simulink model "EkfObserver"  (R2026b)
settings: Solver=VariableStepAuto
PostLoadFcn:
  | addpath(fullfile(fileparts(get_param(bdroot,'FileName')),'..','build_process'));initialize_ekf_paths();
undefined symbols (not defined in the file or in its folder): ekf_parameters
libraries: $bdroot x1
settings Model: Creator=24322  LastModifiedBy=24322

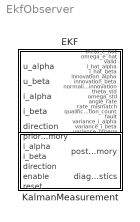
== system EkfObserver ==
  EKF : Subsystem  mask{cfg=ekf_parameters()}
      mask prompts: cfg "Kalman configuration"
  KalmanMeasurement : Subsystem  mask{cfg=ekf_parameters()}
      mask prompts: cfg "Kalman configuration"

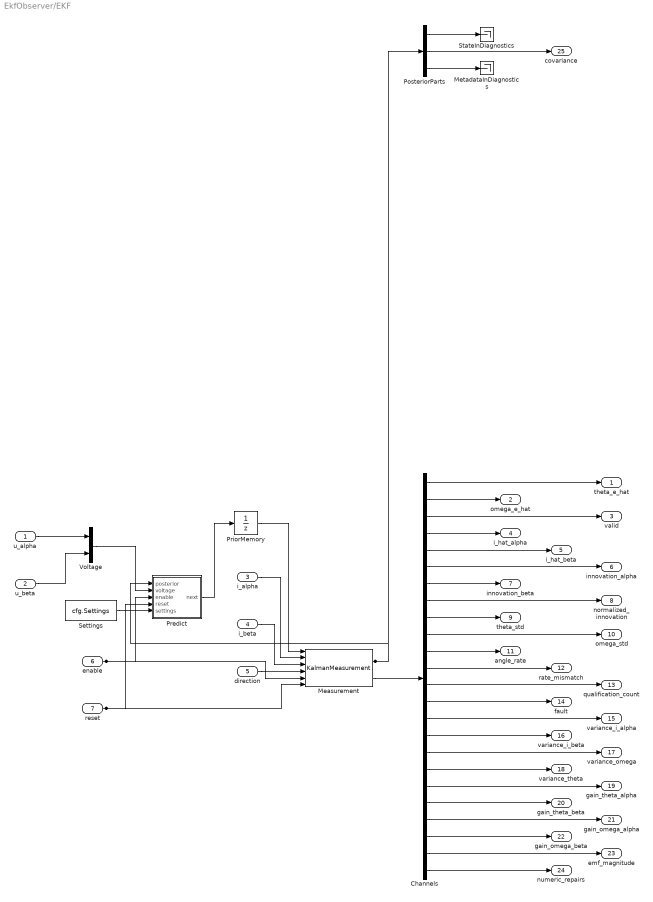
== system EkfObserver/EKF ==
  u_alpha : Inport  SampleTime=cfg.Model.Ts
  u_beta : Inport  Port=2  SampleTime=cfg.Model.Ts
  i_alpha : Inport  Port=3  SampleTime=cfg.Model.Ts
  i_beta : Inport  Port=4  SampleTime=cfg.Model.Ts
  direction : Inport  Port=5  SampleTime=cfg.Model.Ts
  enable : Inport  Port=6  SampleTime=cfg.Model.Ts
  reset : Inport  Port=7  SampleTime=cfg.Model.Ts
  Channels : Demux  Outputs=24
  Measurement : $bdroot/KalmanMeasurement  cfg=cfg
  MetadataInDiagnostics : Terminator
  PosteriorParts : Demux  Outputs=[4 16 8]
  Predict : MATLAB Function  TreatAsAtomicUnit=on
  PriorMemory : UnitDelay  InitialCondition=zeros(28,1)  SampleTime=cfg.Model.Ts
  Settings : Constant  Value=cfg.Settings
  StateInDiagnostics : Terminator
  Voltage : Mux  Inputs=2
  theta_e_hat : Outport
  omega_e_hat : Outport  Port=2
  valid : Outport  Port=3
  i_hat_alpha : Outport  Port=4
  i_hat_beta : Outport  Port=5
  innovation_alpha : Outport  Port=6
  innovation_beta : Outport  Port=7
  normalized_innovation : Outport  Port=8
  theta_std : Outport  Port=9
  omega_std : Outport  Port=10
  angle_rate : Outport  Port=11
  rate_mismatch : Outport  Port=12
  qualification_count : Outport  Port=13
  fault : Outport  Port=14
  variance_i_alpha : Outport  Port=15
  variance_i_beta : Outport  Port=16
  variance_omega : Outport  Port=17
  variance_theta : Outport  Port=18
  gain_theta_alpha : Outport  Port=19
  gain_theta_beta : Outport  Port=20
  gain_omega_alpha : Outport  Port=21
  gain_omega_beta : Outport  Port=22
  emf_magnitude : Outport  Port=23
  numeric_repairs : Outport  Port=24
  covariance : Outport  Port=25
  wires:
  Channels/24 -> numeric_repairs/1
  Channels/23 -> emf_magnitude/1
  Channels/22 -> gain_omega_beta/1
  Channels/21 -> gain_omega_alpha/1
  Channels/20 -> gain_theta_beta/1
  Channels/19 -> gain_theta_alpha/1
  Channels/18 -> variance_theta/1
  Channels/17 -> variance_omega/1
  Channels/16 -> variance_i_beta/1
  Channels/15 -> variance_i_alpha/1
  Channels/14 -> fault/1
  Channels/13 -> qualification_count/1
  Channels/12 -> rate_mismatch/1
  Channels/11 -> angle_rate/1
  Channels/10 -> omega_std/1
  Channels/9 -> theta_std/1
  Channels/8 -> normalized_innovation/1
  Channels/7 -> innovation_beta/1
  Channels/6 -> innovation_alpha/1
  Channels/5 -> i_hat_beta/1
  Channels/4 -> i_hat_alpha/1
  Channels/3 -> valid/1
  Channels/2 -> omega_e_hat/1
  Channels/1 -> theta_e_hat/1
  PosteriorParts/3 -> MetadataInDiagnostics/1
  PosteriorParts/2 -> covariance/1
  PosteriorParts/1 -> StateInDiagnostics/1
  Measurement/2 -> Channels/1
  Predict/1(next) -> PriorMemory/1
  Settings/1 -> Predict/5(settings)
  Voltage/1 -> Predict/2(voltage)
  Measurement/1 -> PosteriorParts/1, Predict/1(posterior)
  reset/1 -> Measurement/6, Predict/4(reset)
  enable/1 -> Measurement/5, Predict/3(enable)
  direction/1 -> Measurement/4
  i_beta/1 -> Measurement/3
  i_alpha/1 -> Measurement/2
  PriorMemory/1 -> Measurement/1
  u_beta/1 -> Voltage/2
  u_alpha/1 -> Voltage/1

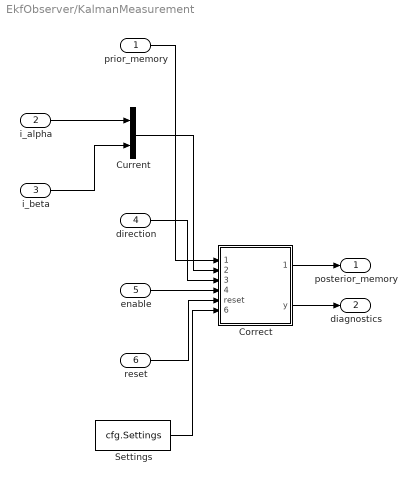
== system EkfObserver/KalmanMeasurement ==
  prior_memory : Inport  PortDimensions=28  SampleTime=cfg.Model.Ts
  i_alpha : Inport  Port=2  SampleTime=cfg.Model.Ts
  i_beta : Inport  Port=3  SampleTime=cfg.Model.Ts
  direction : Inport  Port=4  SampleTime=cfg.Model.Ts
  enable : Inport  Port=5  SampleTime=cfg.Model.Ts
  reset : Inport  Port=6  SampleTime=cfg.Model.Ts
  Correct : MATLAB Function  TreatAsAtomicUnit=on
  Current : Mux  Inputs=2
  Settings : Constant  Value=cfg.Settings
  posterior_memory : Outport
  diagnostics : Outport  Port=2
  wires:
  Correct/2(y) -> diagnostics/1
  Correct/1(posterior) -> posterior_memory/1
  Settings/1 -> Correct/6(settings)
  reset/1 -> Correct/5(reset)
  enable/1 -> Correct/4(enable)
  direction/1 -> Correct/3(direction)
  Current/1 -> Correct/2(current)
  prior_memory/1 -> Correct/1(memory)
  i_beta/1 -> Current/2
  i_alpha/1 -> Current/1

== matlab function EkfObserver/EKF/Predict ==
  data: posterior input; next output; voltage input; enable input; reset input; settings input
function next=ekf_predict(posterior,voltage,enable,reset,settings)
%EKF_PREDICT Advance posterior and covariance to the next current-measurement time.
%#codegen
next=posterior;s=cast(settings,'like',posterior);
if enable<.5 || reset>.5 || posterior(26)>0 || posterior(27)<.5,return;end
applied=cast(voltage,'like',posterior);
if ~all(isfinite(applied)) || any(abs(applied)>s(27))
    next(26)=1;next(21)=0;next(3)=0;return;
end
if abs(posterior(3))>s(25)
    next(26)=3;next(21)=0;next(3)=0;return;
end
[state,a]=pmsm_sensorless_step(posterior(1:4),applied,s(1:4));
p=reshape(posterior(5:20),4,4);p=a*p*a'+diag(s(11:14));p=.5*(p+p');
if ~all(isfinite(state)) || ~all(isfinite(p),'all') || any(diag(p)<0)
    next(26)=3;next(21)=0;next(3)=0;return;
end
next(1:4)=state;next(5:20)=p(:);
end

== matlab function EkfObserver/KalmanMeasurement/Correct ==
  data: posterior output; memory input; y output; current input; direction input; enable input; reset input; settings input
function [posterior,y]=kalman_current_update(memory,current,direction,enable,reset,settings)
%KALMAN_CURRENT_UPDATE Shared four-state current correction and qualification.
% memory=[prior x(4);prior P(:)(16);count;previous theta;angle rate;have theta;
%         previous direction;fault;initialized;numeric repair count].
% The current measurement is used now; current voltage is not an input.
%#codegen
s=cast(settings,'like',memory);posterior=zeros(28,1,'like',memory);y=zeros(24,1,'like',memory);
validSettings=all(isfinite(s)) && s(1)>0 && s(2)>=0 && s(3)>0 && s(4)>0 && ...
    all(s(7:16)>0) && s(17)>=1 && all(s(18:22)>0) && s(23)>0 && s(23)<=1 && all(s(24:27)>0);
if ~validSettings,posterior(26)=2;y(14)=2;return;end
posterior=initial_pack(s,memory);
innovation=zeros(2,1,'like',memory);gain=zeros(4,2,'like',memory);nis=cast(0,'like',memory);
if (isfinite(reset) && reset>.5) || (isfinite(enable) && enable<.5)
    y=outputs(posterior,innovation,nis,gain,s);return;
end
if ~isfinite(enable) || ~isfinite(reset) || ~isfinite(direction) || (direction~=0 && abs(direction)~=1)
    posterior(26)=2;y=outputs(posterior,innovation,nis,gain,s);return;
end
if ~all(isfinite(memory))
    posterior(26)=3;y=outputs(posterior,innovation,nis,gain,s);return;
end
if memory(26)>0
    posterior=memory;posterior(21)=0;posterior(3)=0;
    y=outputs(posterior,innovation,nis,gain,s);return;
end
measured=cast(current,'like',memory);
if ~all(isfinite(measured)) || any(abs(measured)>s(26))
    if memory(27)>.5,posterior=memory;end
    posterior(26)=1;posterior(21)=0;posterior(3)=0;
    y=outputs(posterior,innovation,nis,gain,s);return;
end
if memory(27)>.5
    prior=memory(1:4);covariance=reshape(memory(5:20),4,4);posterior=memory;
else
    prior=posterior(1:4);prior(3)=direction*s(5);
    covariance=reshape(posterior(5:20),4,4);
end
[predictedMeasurement,h]=pmsm_sensorless_measurement(prior);
innovation=measured-predictedMeasurement;r=diag(s(15:16));
innovationCov=h*covariance*h'+r;determinant=innovationCov(1,1)*innovationCov(2,2)-innovationCov(1,2)*innovationCov(2,1);
if ~all(isfinite(innovationCov),'all') || any(diag(innovationCov)<=0) || ~isfinite(determinant) || determinant<=0
    posterior=initial_pack(s,memory);posterior(26)=3;y=outputs(posterior,zeros(2,1,'like',memory),nis,gain,s);return;
end
gain=(covariance*h')/innovationCov;state=prior+gain*innovation;
state(4)=atan2(sin(state(4)),cos(state(4)));
nis=innovation'*(innovationCov\innovation);
identity=eye(4,'like',memory);m=identity-gain*h;
covariance=m*covariance*m'+gain*r*gain';covariance=.5*(covariance+covariance');
if ~all(isfinite(state)) || ~all(isfinite(covariance),'all') || any(diag(covariance)<0) || ~isfinite(nis) || nis<0
    posterior=initial_pack(s,memory);posterior(26)=3;y=outputs(posterior,zeros(2,1,'like',memory),cast(0,'like',memory),zeros(4,2,'like',memory),s);return;
end
if memory(24)>.5
    difference=atan2(sin(state(4)-memory(22)),cos(state(4)-memory(22)));
    rate=memory(23)+s(23)*(difference/s(1)-memory(23));
else
    rate=state(3);
end
count=cast(0,'like',memory);
qualified=direction~=0 && direction*state(3)>=s(18) && abs(state(3))<=s(25) && abs(state(3))*s(4)>=s(19) && ...
    nis<=s(20) && sqrt(covariance(4,4))<=s(21) && sqrt(covariance(3,3))<=s(22) && abs(rate-state(3))<=s(24);
if qualified
    if direction==memory(25),count=min(memory(21)+1,s(17));else,count=cast(1,'like',memory);end
end
posterior(1:4)=state;posterior(5:20)=covariance(:);posterior(21)=count;
posterior(22)=state(4);posterior(23)=rate;posterior(24)=1;
posterior(25)=direction;posterior(26)=0;posterior(27)=1;posterior(28)=memory(28);
y=outputs(posterior,innovation,nis,gain,s);
end
function pack=initial_pack(s,like)
pack=zeros(28,1,'like',like);pack(4)=s(6);p=diag(s(7:10));pack(5:20)=p(:);
end
function y=outputs(pack,innovation,nis,gain,s)
y=zeros(24,1,'like',pack);p=reshape(pack(5:20),4,4);
y(1)=pack(4);y(2)=pack(3);y(3)=cast(pack(21)>=s(17) && pack(26)==0,'like',pack);
y(4:5)=pack(1:2);y(6:7)=innovation;y(8)=nis;
y(9)=sqrt(max(p(4,4),0));y(10)=sqrt(max(p(3,3),0));
y(11)=pack(23);y(12)=pack(23)-pack(3);y(13)=pack(21);y(14)=pack(26);
y(15:18)=diag(p);y(19:20)=gain(4,:)';y(21:22)=gain(3,:)';y(23)=abs(pack(3))*s(4);y(24)=pack(28);
end
